simulink model "TV_FLC_V3"  (R2026b)
settings: Solver=VariableStepAuto
model mask{MotorT=Control.MotorTrq, Gr=Control.GearRatio, MotorW=Control.MotorW, rwheel=Control.WheelRad, tr=Control.RearTrack, a=Control.FrontTrackToCG, a_cop=Control.FrontTrackToCoP, Af=Control.FrontalArea, cd=Control.LiftCoef, Value=Control.GravitationalAcc, ro=Control.AirDensity, m=Control.Mass, h_CG=Control.CGHeight, L=Control.Wheelbase, StrWhlR=Control.StrWheelRatio, Ku=Control.UndersteerGradient, F=Control.F, Slip_Ctrl_Kp=Control.Proportional_P, Slip_Ctrl_Ki=Control.Integral_I, Slip_Ctrl_Kd=Control.Derivative_D, Slip_Ctrl_Kn=Control.Filter_N, Load_Ref=Control.LoadRef, Slip_Ref=Control.SlipRef, FIS=Control.FuzzySystem, vx_th=Control.ActivationVelocity, Tmax=max(Control.MotorTrq), C_alpha_F=Control.CalphaF, Slip_Steer_th=10, Kp_TV_Yaw=Control.Kp_Yaw, Kp_TV_Beta=Control.Kp_beta}
  mask prompts: MotorT "Motor Torque:"; Gr "Gear Ratio:"; MotorW "Motor RPM:"; rwheel "Wheel Radius:"; tr "Rear Track:"; a "Front Track to CG:"; a_cop "Front Track to CoP"; Af "Frontal Area:"; cd "Lift Coef:"; Value "Simulink:blkprm_prompts:ConstConstValue"; ro "Air Density:"; m "Mass:"; h_CG "CG Height:"; L "Wheelbase:"; StrWhlR "Steering Wheel Ratio:"; Ku "Understeer Gradient:"; F "Moment to Torque"; Slip_Ctrl_Kp "Simulink:masks:ProportionalP_MP"; Slip_Ctrl_Ki "Simulink:masks:IntegralI_MP"; Slip_Ctrl_Kd "Simulink:masks:DerivativeD_MP"; Slip_Ctrl_Kn "Filter (N):"; Load_Ref "Reference Load Table:"; Slip_Ref "Reference Slip Table:"; FIS "Fuzzy Inference System"; vx_th "Activation Velocity:"; Tmax "Max Torque"; C_alpha_F "Front Cornering Stiffness:"; Slip_Steer_th "Steering activation threshold:"; Kp_TV_Yaw "TV Yaw factor:"; Kp_TV_Beta "TV Beta factor:"
values from neighbouring files (symbols this model uses):
  a = -Vehicle.Chassis.Body.sCG.Value(1)    [sm_car_controlparam_FLCDYC_V3.m]
  Gr = 1/Vehicle.Powertrain.Driveline.Gearbox.ratio.Value    [sm_car_controlparam_FLCDYC_V3.m]
  L = 1.578    [sm_car_controlparam_FLCDYC_V3.m]
  rwheel = 0.263    [sm_car_controlparam_FLCDYC_V3.m]
  tr = Vehicle.Chassis.Body.TrackRear.Value    [sm_car_controlparam_FLCDYC_V3.m]
undefined symbols (not defined in the file or in its folder): dspblkCoreblockFVToolHelper, gcbh
libraries: simulink x5, sl_discontinuities x3, slpidlib x2, fuzblock x1
settings Model: Creator=andrei  LastModifiedBy=andrei

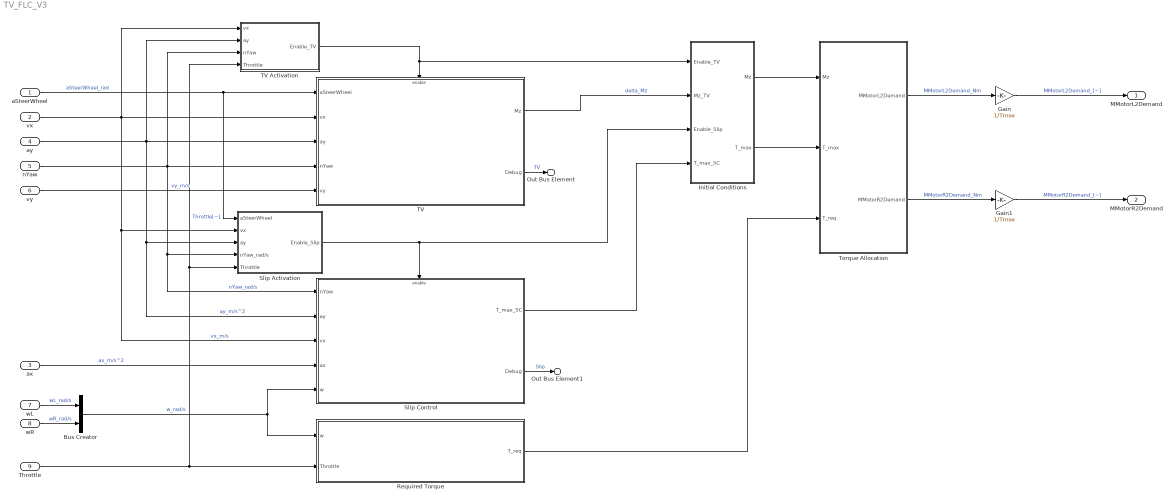
== system TV_FLC_V3 ==
  aSteerWheel : Inport  OutDataTypeStr=single  PortDimensions=1  SampleTime=0.003
  vx : Inport  Port=2  OutDataTypeStr=single  PortDimensions=1  SampleTime=0.003
  ax : Inport  Port=3  OutDataTypeStr=single  PortDimensions=1  SampleTime=0.003
  ay : Inport  Port=4  OutDataTypeStr=single  PortDimensions=1  SampleTime=0.003
  nYaw : Inport  Port=5  OutDataTypeStr=single  PortDimensions=1  SampleTime=0.003
  vy : Inport  Port=6  OutDataTypeStr=single  PortDimensions=1  SampleTime=0.003
  wL : Inport  Port=7  OutDataTypeStr=single  PortDimensions=1  SampleTime=0.003
  wR : Inport  Port=8  OutDataTypeStr=single  PortDimensions=1  SampleTime=0.003
  Throttle : Inport  Port=9  OutDataTypeStr=single  PortDimensions=1  SampleTime=0.003
  Bus Creator : BusCreator  Inputs=2
  Gain : Gain  Gain=1/Tmax
  Gain1 : Gain  Gain=1/Tmax
  Initial Conditions : Subsystem
  Required Torque : Subsystem
  Slip Activation : Subsystem
  Slip Control : Subsystem
  TV : Subsystem
  TV Activation : Subsystem
  Torque Allocation : Subsystem
  MMotorL2Demand : Outport  OutDataTypeStr=single  PortDimensions=1  SampleTime=0.003
  MMotorR2Demand : Outport  Port=2  OutDataTypeStr=single  PortDimensions=1  SampleTime=0.003
  Out Bus Element : Outport  Port=3  PortName=Debug  Element=TV
  Out Bus Element1 : Outport  Port=3  PortName=Debug  Element=Slip
  wires:
  Gain1/1 -> MMotorR2Demand/1  "MMotorR2Demand_[~]"
  Torque Allocation/2(MMotorR2Demand) -> Gain1/1  "MMotorR2Demand_Nm"
  vy/1 -> TV/5(vy)  "vy_m/s"
  Gain/1 -> MMotorL2Demand/1  "MMotorL2Demand_[~]"
  Slip Control/1(T_max_SC) -> Initial Conditions/4(T_max_SC)
  Slip Control/2(Debug) -> Out Bus Element1/1  "Slip"
  ax/1 -> Slip Control/4(ax)  "ax_m/s^2"
  Initial Conditions/2(T_max) -> Torque Allocation/2(T_max)
  wL/1 -> Bus Creator/1  "wL_rad/s"
  TV/1(Mz) -> Initial Conditions/2(Mz_TV)  "delta_Mz"
  Torque Allocation/1(MMotorL2Demand) -> Gain/1  "MMotorL2Demand_Nm"
  TV Activation/1(Enable_TV) -> Initial Conditions/1(Enable_TV), TV/Enable
  TV/2(Debug) -> Out Bus Element/1  "TV"
  wR/1 -> Bus Creator/2  "wR_rad/s"
  Bus Creator/1 -> Required Torque/1(w), Slip Control/5(w)  "w_rad/s"
  Initial Conditions/1(Mz) -> Torque Allocation/1(Mz)
  Required Torque/1(T_req) -> Torque Allocation/3(T_req)
  vx/1 -> TV Activation/1(vx), Slip Activation/2(vx), Slip Control/3(vx), TV/2(vx)  "vx_m/s"
  nYaw/1 -> TV Activation/3(nYaw), TV/4(nYaw), Slip Activation/4(nYaw_rad/s), Slip Control/1(nYaw)  "nYaw_rad/s"
  Throttle/1 -> TV Activation/4(Throttle), Slip Activation/5(Throttle), Required Torque/2(Throttle)  "Throttle[~]"
  aSteerWheel/1 -> Slip Activation/1(aSteerWheel), TV/1(aSteerWheel)  "aSteerWheel_rad"
  ay/1 -> Slip Activation/3(ay), Slip Control/2(ay), TV Activation/2(ay), TV/3(ay)  "ay_m/s^2"
  Slip Activation/1(Enable_Slip) -> Slip Control/Enable, Initial Conditions/3(Enable_Slip)

== system TV_FLC_V3/Initial Conditions ==
  Enable_TV : Inport
  Mz_TV : Inport  Port=2
  Enable_Slip : Inport  Port=3
  T_max_SC : Inport  Port=4
  Bus Creator1 : BusCreator  Inputs=2
  Constant : Constant  Value=Tmax  OutDataTypeStr=single
  Constant1 : Constant  Value=Tmax  OutDataTypeStr=single
  Constant2 : Constant  Value=0  OutDataTypeStr=single
  Switch : Switch  Criteria=u2 ~= 0  SaturateOnIntegerOverflow=off  InputSameDT=off
  Switch1 : Switch  Criteria=u2 ~= 0  SaturateOnIntegerOverflow=off  InputSameDT=off
  Mz : Outport
  T_max : Outport  Port=2
  wires:
  Enable_Slip/1 -> Switch/2
  Enable_TV/1 -> Switch1/2
  Constant1/1 -> Bus Creator1/2  "Tmax_rr_Nm"
  Switch/1 -> T_max/1
  Bus Creator1/1 -> Switch/3
  T_max_SC/1 -> Switch/1
  Constant/1 -> Bus Creator1/1  "Tmax_rl_Nm"
  Mz_TV/1 -> Switch1/1
  Constant2/1 -> Switch1/3  "Mz"
  Switch1/1 -> Mz/1

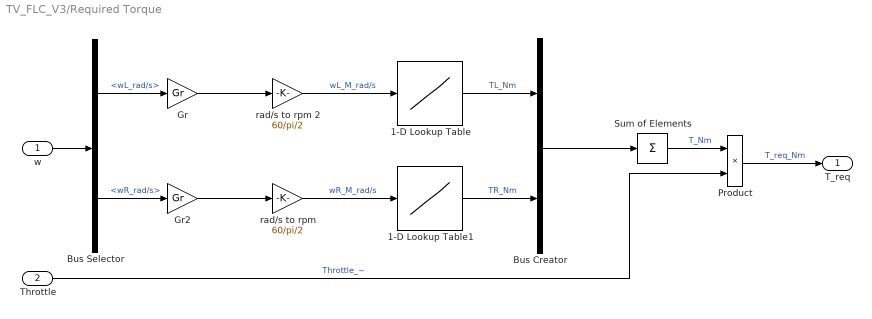
== system TV_FLC_V3/Required Torque ==
  w : Inport
  Throttle : Inport  Port=2
  1-D Lookup Table : Lookup_n-D  NumberOfTableDimensions=1  BreakpointsForDimension1=MotorW  Table=MotorT  InternalRulePriority=Speed  RndMeth=Simplest
  1-D Lookup Table1 : Lookup_n-D  NumberOfTableDimensions=1  BreakpointsForDimension1=MotorW  Table=MotorT  InternalRulePriority=Speed  RndMeth=Simplest
  Bus Creator : BusCreator  Inputs=2
  Bus Selector : BusSelector  OutputSignals=wL_rad/s,wR_rad/s
  Gr : Gain  Gain=Gr
  Gr2 : Gain  Gain=Gr
  Product : Product
  Sum of Elements : Sum  Inputs=+
  rad/s to rpm : Gain  Gain=60/pi/2
  rad/s to rpm 2 : Gain  Gain=60/pi/2
  T_req : Outport
  wires:
  w/1 -> Bus Selector/1
  Sum of Elements/1 -> Product/1  "T_Nm"
  1-D Lookup Table1/1 -> Bus Creator/2  "TR_Nm"
  Throttle/1 -> Product/2  "Throttle_~"
  rad/s to rpm/1 -> 1-D Lookup Table1/1  "wR_M_rad/s"
  Bus Selector/1 -> Gr/1  "<wL_rad/s>"
  Product/1 -> T_req/1  "T_req_Nm"
  Bus Selector/2 -> Gr2/1  "<wR_rad/s>"
  rad/s to rpm 2/1 -> 1-D Lookup Table/1  "wL_M_rad/s"
  1-D Lookup Table/1 -> Bus Creator/1  "TL_Nm"
  Bus Creator/1 -> Sum of Elements/1
  Gr/1 -> rad/s to rpm 2/1
  Gr2/1 -> rad/s to rpm/1

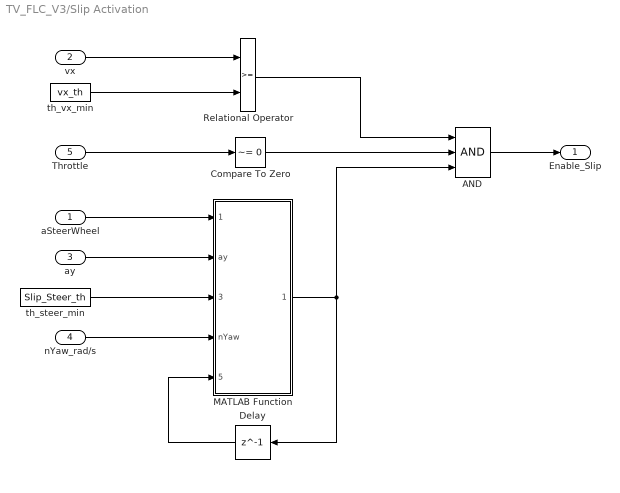
== system TV_FLC_V3/Slip Activation ==
  aSteerWheel : Inport
  vx : Inport  Port=2
  ay : Inport  Port=3
  nYaw_rad/s : Inport  Port=4
  Throttle : Inport  Port=5
  AND : Logic  Inputs=3  AllPortsSameDT=off  OutDataTypeStr=boolean
  Compare To Zero : simulink/Logic and Bit Operations/Compare To Zero  relop=~=  OutDataTypeStr=boolean
  Delay : Delay  DelayLength=1
  MATLAB Function : MATLAB Function  TreatAsAtomicUnit=on
  Relational Operator : RelationalOperator  OutDataTypeStr=boolean  RndMeth=Simplest  InputSameDT=off
  th_steer_min : Constant  Value=Slip_Steer_th
  th_vx_min : Constant  Value=vx_th
  Enable_Slip : Outport
  wires:
  Compare To Zero/1 -> AND/2
  AND/1 -> Enable_Slip/1
  Throttle/1 -> Compare To Zero/1
  th_vx_min/1 -> Relational Operator/2
  vx/1 -> Relational Operator/1
  Relational Operator/1 -> AND/1
  aSteerWheel/1 -> MATLAB Function/1(aSteerWheel)
  th_steer_min/1 -> MATLAB Function/3(steer_th)
  ay/1 -> MATLAB Function/2(ay)
  nYaw_rad/s/1 -> MATLAB Function/4(nYaw)
  MATLAB Function/1(slip_active) -> Delay/1, AND/3
  Delay/1 -> MATLAB Function/5(slip_active_previous)

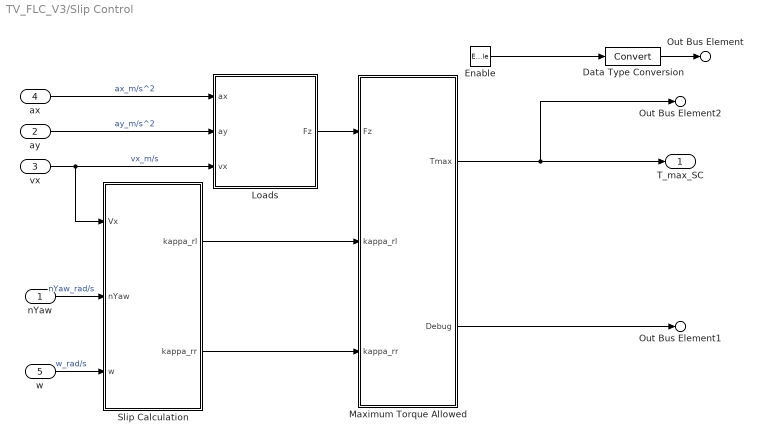
== system TV_FLC_V3/Slip Control ==
  nYaw : Inport
  ay : Inport  Port=2
  vx : Inport  Port=3
  ax : Inport  Port=4
  w : Inport  Port=5
  Enable : EnablePort  StatesWhenEnabling=reset  ShowOutputPort=on  OutDataTypeStr=boolean
  Data Type Conversion : DataTypeConversion  SaturateOnIntegerOverflow=off  RndMeth=Floor
  Loads : Subsystem
  Maximum Torque Allowed : Subsystem
  Slip Calculation : Subsystem
  T_max_SC : Outport  OutputWhenDisabled=reset  InitialOutput=Tmax
  Out Bus Element : Outport  Port=2  PortName=Debug  Element=State
  Out Bus Element1 : Outport  Port=2  PortName=Debug  Element=Controller
  Out Bus Element2 : Outport  Port=2  PortName=Debug  Element=TmaxOut
  wires:
  Maximum Torque Allowed/2(Debug) -> Out Bus Element1/1
  Enable/1 -> Data Type Conversion/1
  w/1 -> Slip Calculation/3(w)  "w_rad/s"
  nYaw/1 -> Slip Calculation/2(nYaw)  "nYaw_rad/s"
  ax/1 -> Loads/1(ax)  "ax_m/s^2"
  Loads/1(Fz) -> Maximum Torque Allowed/1(Fz)
  ay/1 -> Loads/2(ay)  "ay_m/s^2"
  Slip Calculation/2(kappa_rr) -> Maximum Torque Allowed/3(kappa_rr)
  vx/1 -> Loads/3(vx), Slip Calculation/1(Vx)  "vx_m/s"
  Slip Calculation/1(kappa_rl) -> Maximum Torque Allowed/2(kappa_rl)
  Data Type Conversion/1 -> Out Bus Element/1
  Maximum Torque Allowed/1(Tmax) -> Out Bus Element2/1, T_max_SC/1

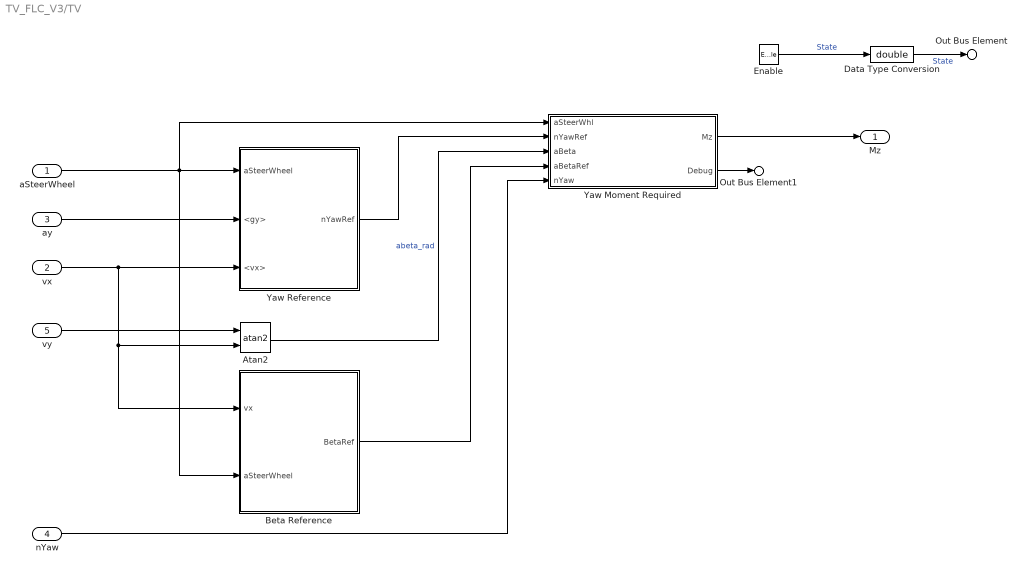
== system TV_FLC_V3/TV ==
  aSteerWheel : Inport
  vx : Inport  Port=2
  ay : Inport  Port=3
  nYaw : Inport  Port=4
  vy : Inport  Port=5
  Enable : EnablePort  StatesWhenEnabling=reset  ShowOutputPort=on  OutDataTypeStr=boolean
  Atan2 : Trigonometry  Operator=atan2
  Beta Reference : Subsystem
  Data Type Conversion : DataTypeConversion  OutDataTypeStr=double  SaturateOnIntegerOverflow=off  RndMeth=Floor
  Yaw Moment Required : Subsystem
  Yaw Reference : Subsystem
  Mz : Outport  OutputWhenDisabled=reset  InitialOutput=0
  Out Bus Element : Outport  Port=2  PortName=Debug  Element=State
  Out Bus Element1 : Outport  Port=2  PortName=Debug  Element=Controller
  wires:
  Yaw Moment Required/2(Debug) -> Out Bus Element1/1
  Data Type Conversion/1 -> Out Bus Element/1  "State"
  vy/1 -> Atan2/1
  Beta Reference/1(BetaRef) -> Yaw Moment Required/4(aBetaRef)
  Yaw Reference/1(nYawRef) -> Yaw Moment Required/2(nYawRef)
  ay/1 -> Yaw Reference/2(<gy>)
  nYaw/1 -> Yaw Moment Required/5(nYaw)
  vx/1 -> Yaw Reference/3(<vx>), Atan2/2, Beta Reference/1(vx)
  aSteerWheel/1 -> Yaw Reference/1(aSteerWheel), Yaw Moment Required/1(aSteerWhl), Beta Reference/2(aSteerWheel)
  Atan2/1 -> Yaw Moment Required/3(aBeta)  "abeta_rad"
  Yaw Moment Required/1(Mz) -> Mz/1
  Enable/1 -> Data Type Conversion/1  "State"

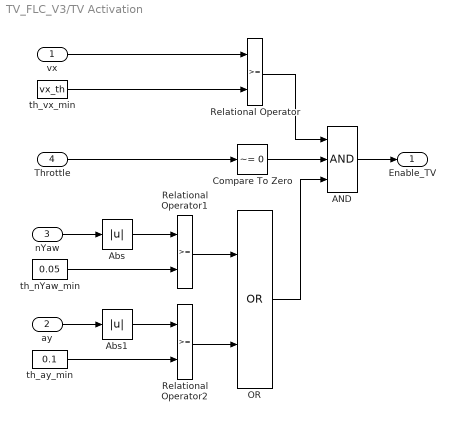
== system TV_FLC_V3/TV Activation ==
  vx : Inport
  ay : Inport  Port=2
  nYaw : Inport  Port=3
  Throttle : Inport  Port=4
  AND : Logic  Inputs=3  AllPortsSameDT=off  OutDataTypeStr=boolean
  Abs : Abs  SaturateOnIntegerOverflow=off
  Abs1 : Abs  SaturateOnIntegerOverflow=off
  Compare To Zero : simulink/Logic and Bit Operations/Compare To Zero  relop=~=  OutDataTypeStr=boolean
  OR : Logic  Operator=OR  AllPortsSameDT=off  OutDataTypeStr=boolean
  Relational Operator : RelationalOperator  OutDataTypeStr=boolean  RndMeth=Simplest  InputSameDT=off
  Relational Operator1 : RelationalOperator  OutDataTypeStr=boolean  RndMeth=Simplest  InputSameDT=off
  Relational Operator2 : RelationalOperator  OutDataTypeStr=boolean  RndMeth=Simplest  InputSameDT=off
  th_ay_min : Constant  Value=0.1  OutDataTypeStr=single
  th_nYaw_min : Constant  Value=0.05  OutDataTypeStr=single
  th_vx_min : Constant  Value=vx_th
  Enable_TV : Outport
  wires:
  ay/1 -> Abs1/1
  th_nYaw_min/1 -> Relational Operator1/2
  Abs1/1 -> Relational Operator2/1
  Throttle/1 -> Compare To Zero/1
  Abs/1 -> Relational Operator1/1
  vx/1 -> Relational Operator/1
  nYaw/1 -> Abs/1
  th_ay_min/1 -> Relational Operator2/2
  th_vx_min/1 -> Relational Operator/2
  Relational Operator1/1 -> OR/1
  Relational Operator2/1 -> OR/2
  Relational Operator/1 -> AND/1
  Compare To Zero/1 -> AND/2
  OR/1 -> AND/3
  AND/1 -> Enable_TV/1

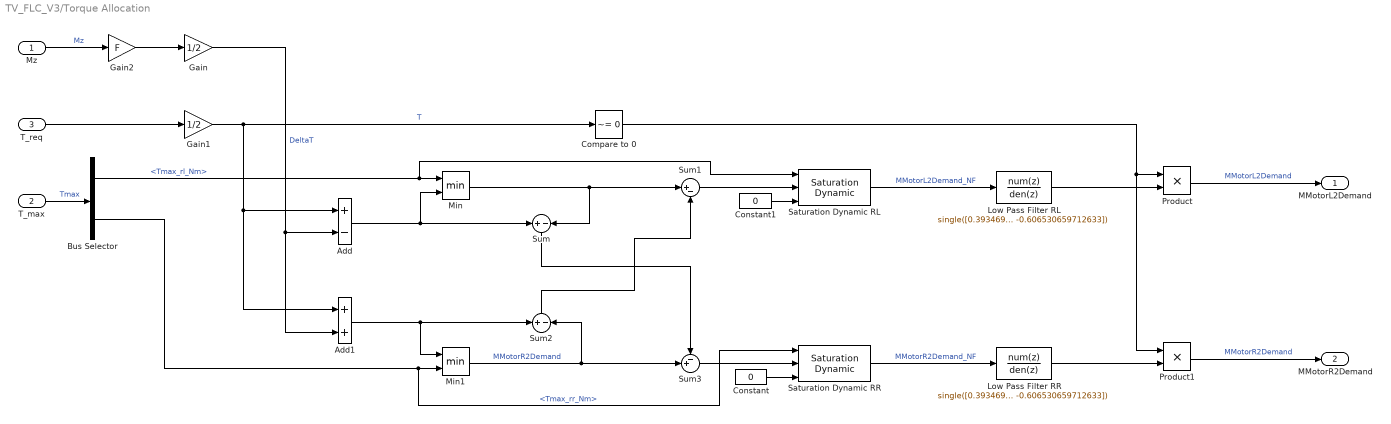
== system TV_FLC_V3/Torque Allocation ==
  Mz : Inport
  T_max : Inport  Port=2
  T_req : Inport  Port=3
  Add : Sum  Inputs=+-
  Add1 : Sum
  Bus Selector : BusSelector  OutputSignals=Tmax_rl_Nm,Tmax_rr_Nm
  "Compare to 0 " : simulink/Logic and Bit Operations/Compare To Constant  relop=~=  const=0  OutDataTypeStr=boolean
  Constant : Constant  Value=0
  Constant1 : Constant  Value=0
  Gain : Gain  Gain=1/2
  Gain1 : Gain  Gain=1/2
  Gain2 : Gain  Gain=F
  Low Pass Filter RL : DiscreteTransferFcn  LoadFcn=dspblkCoreblockFVToolHelper(gcbh,'load');  Numerator=single([0.393469340287367])  Denominator=single([1 -0.606530659712633])
      settings: CopyFcn=dspblkCoreblockFVToolHelper(gcbh,'copy');  DeleteFcn=dspblkCoreblockFVToolHelper(gcbh,'close');  ModelCloseFcn=dspblkCoreblockFVToolHelper(gcbh,'close');  PreSaveFcn=dspblkCoreblockFVToolHelper(gcbh,'presave');  PostSaveFcn=dspblkCoreblockFVToolHelper(gcbh,'postsave');  CloseFcn=dspblkCoreblockFVToolHelper(gcbh,'close');
  Low Pass Filter RR : DiscreteTransferFcn  LoadFcn=dspblkCoreblockFVToolHelper(gcbh,'load');  Numerator=single([0.393469340287367])  Denominator=single([1 -0.606530659712633])
      settings: CopyFcn=dspblkCoreblockFVToolHelper(gcbh,'copy');  DeleteFcn=dspblkCoreblockFVToolHelper(gcbh,'close');  ModelCloseFcn=dspblkCoreblockFVToolHelper(gcbh,'close');  PreSaveFcn=dspblkCoreblockFVToolHelper(gcbh,'presave');  PostSaveFcn=dspblkCoreblockFVToolHelper(gcbh,'postsave');  CloseFcn=dspblkCoreblockFVToolHelper(gcbh,'close');
  Min : MinMax  Inputs=2
  Min1 : MinMax  Inputs=2
  Product : Product
  Product1 : Product
  Saturation Dynamic RL : sl_discontinuities/Saturation Dynamic  OutMin=[]  OutMax=[]  OutDataTypeStr=single  OutDataType=fixdt(1, 16)  OutScaling=2^-10  DoSatur=off
      settings: LibrarySourceBlock=|
      | simulink/Discontinuities/Saturation
      | Dynamic
  Saturation Dynamic RR : sl_discontinuities/Saturation Dynamic  OutMin=[]  OutMax=[]  OutDataTypeStr=single  OutDataType=fixdt(1, 16)  OutScaling=2^-10  DoSatur=off
      settings: LibrarySourceBlock=|
      | simulink/Discontinuities/Saturation
      | Dynamic
  Sum : Sum  Inputs=+|-
  Sum1 : Sum  Inputs=|+-
  Sum2 : Sum  Inputs=+|-
  Sum3 : Sum  Inputs=-+|
  MMotorL2Demand : Outport
  MMotorR2Demand : Outport  Port=2
  wires:
  Constant1/1 -> Saturation Dynamic RL/3
  Constant/1 -> Saturation Dynamic RR/3
  Product1/1 -> MMotorR2Demand/1  "MMotorR2Demand"
  Low Pass Filter RR/1 -> Product1/2
  Saturation Dynamic RR/1 -> Low Pass Filter RR/1  "MMotorR2Demand_NF"
  Product/1 -> MMotorL2Demand/1  "MMotorL2Demand"
  Low Pass Filter RL/1 -> Product/2
  "Compare to 0 "/1 -> Product1/1, Product/1
  Gain1/1 -> Add/1, Add1/1, "Compare to 0 "/1  "T"
  Sum/1 -> Sum3/1
  Sum2/1 -> Sum1/2
  Add1/1 -> Min1/1, Sum2/1
  Add/1 -> Min/2, Sum/1
  Bus Selector/2 -> Saturation Dynamic RR/1, Min1/2  "<Tmax_rr_Nm>"
  Bus Selector/1 -> Min/1, Saturation Dynamic RL/1  "<Tmax_rl_Nm>"
  T_max/1 -> Bus Selector/1  "Tmax"
  Min1/1 -> Sum3/2, Sum2/2  "MMotorR2Demand"
  Min/1 -> Sum/2, Sum1/1
  Mz/1 -> Gain2/1  "Mz"
  T_req/1 -> Gain1/1
  Gain/1 -> Add/2, Add1/2  "DeltaT"
  Gain2/1 -> Gain/1
  Sum1/1 -> Saturation Dynamic RL/2
  Sum3/1 -> Saturation Dynamic RR/2
  Saturation Dynamic RL/1 -> Low Pass Filter RL/1  "MMotorL2Demand_NF"

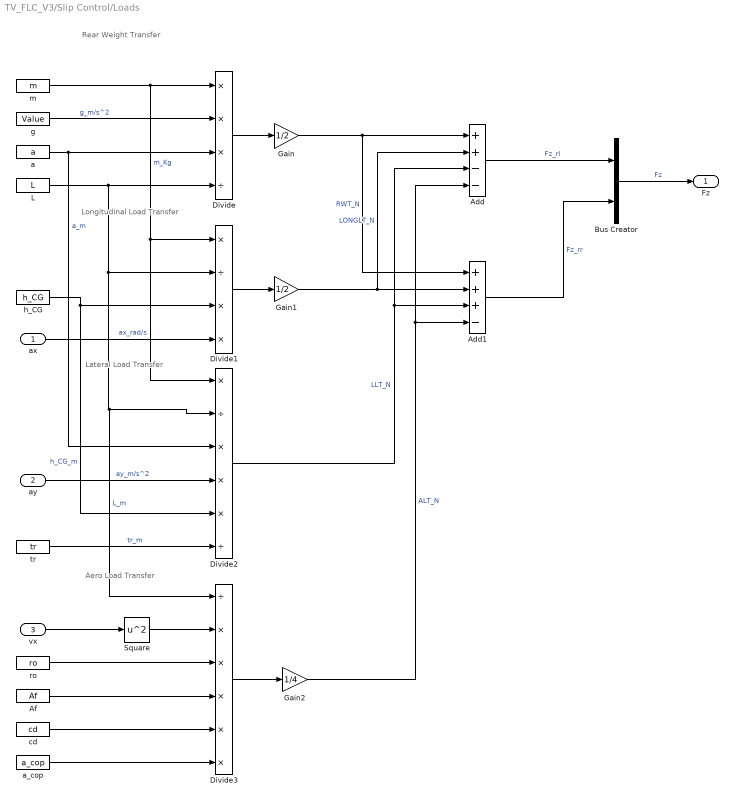
== system TV_FLC_V3/Slip Control/Loads ==
  note: Rear Weight Transfer
  note: Longitudinal Load Transfer
  note: Lateral Load Transfer
  note: Aero Load Transfer
  ax : Inport
  ay : Inport  Port=2
  vx : Inport  Port=3
  Add : Sum  Inputs=++--
  Add1 : Sum  Inputs=+++-
  Af : Constant  Value=Af  OutDataTypeStr=single
  Bus Creator : BusCreator  Inputs=2
  Divide : Product  Inputs=***/
  Divide1 : Product  Inputs=*/**
  Divide2 : Product  Inputs=*/***/
  Divide3 : Product  Inputs=/*****
  Gain : Gain  Gain=1/2
  Gain1 : Gain  Gain=1/2
  Gain2 : Gain  Gain=1/4
  L : Constant  Value=L  OutDataTypeStr=single
  Square : Math  Operator=square
  a : Constant  Value=a  OutDataTypeStr=single
  a_cop : Constant  Value=a_cop  OutDataTypeStr=single
  cd : Constant  Value=cd  OutDataTypeStr=single
  g : Constant  Value=Value  OutDataTypeStr=single
  h_CG : Constant  Value=h_CG  OutDataTypeStr=single
  m : Constant  Value=m  OutDataTypeStr=single
  ro : Constant  Value=ro  OutDataTypeStr=single
  tr : Constant  Value=tr  OutDataTypeStr=single
  Fz : Outport
  wires:
  a_cop/1 -> Divide3/6
  cd/1 -> Divide3/5
  Af/1 -> Divide3/4
  ro/1 -> Divide3/3
  Divide3/1 -> Gain2/1
  Bus Creator/1 -> Fz/1  "Fz"
  Add1/1 -> Bus Creator/2  "Fz_rr"
  Add/1 -> Bus Creator/1  "Fz_rl"
  Divide2/1 -> Add1/3, Add/3  "LLT_N"
  tr/1 -> Divide2/6  "tr_m"
  ay/1 -> Divide2/4  "ay_m/s^2"
  Gain1/1 -> Add1/2, Add/2  "LONGLT_N"
  Divide1/1 -> Gain1/1
  ax/1 -> Divide1/4  "ax_rad/s"
  h_CG/1 -> Divide1/3, Divide2/5  "h_CG_m"
  Gain2/1 -> Add1/4, Add/4  "ALT_N"
  Gain/1 -> Add1/1, Add/1  "RWT_N"
  Square/1 -> Divide3/2
  vx/1 -> Square/1
  Divide/1 -> Gain/1
  L/1 -> Divide/4, Divide1/2, Divide2/2, Divide3/1  "L_m"
  a/1 -> Divide2/3, Divide/3  "a_m"
  g/1 -> Divide/2  "g_m/s^2"
  m/1 -> Divide2/1, Divide1/1, Divide/1  "m_Kg"

== system TV_FLC_V3/Slip Control/Maximum Torque Allowed ==
  Fz : Inport
  kappa_rl : Inport  Port=2
  kappa_rr : Inport  Port=3
  Bus Creator : BusCreator  Inputs=2
  Bus Selector : BusSelector  OutputSignals=Fz_rl,Fz_rr
  Slip Correction Left : Subsystem
  Slip Correction Right : Subsystem
  Tmax : Outport  OutDataTypeStr=single
  Out Bus Element : Outport  Port=2  PortName=Debug  Element=PID_rl
  Out Bus Element1 : Outport  Port=2  PortName=Debug  Element=PID_rr
  wires:
  Slip Correction Right/1(Debug) -> Out Bus Element1/1
  Slip Correction Left/2(Debug) -> Out Bus Element/1
  Slip Correction Right/2(Tmax_rr) -> Bus Creator/2  "Tmax_rr_Nm"
  Slip Correction Left/1(Tmax_rl) -> Bus Creator/1  "Tmax_rl_Nm"
  kappa_rl/1 -> Slip Correction Left/1(kappa_rl)
  kappa_rr/1 -> Slip Correction Right/2(kappa_rr)
  Fz/1 -> Bus Selector/1
  Bus Selector/1 -> Slip Correction Left/2(Fz_rl)  "<Fz_rl>"
  Bus Selector/2 -> Slip Correction Right/1(Fz_rl)  "<Fz_rr>"
  Bus Creator/1 -> Tmax/1

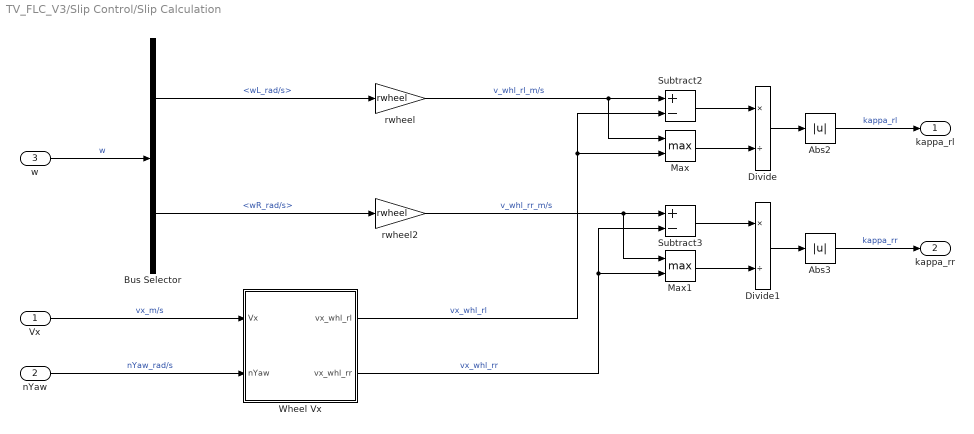
== system TV_FLC_V3/Slip Control/Slip Calculation ==
  Vx : Inport
  nYaw : Inport  Port=2
  w : Inport  Port=3
  Abs2 : Abs  SaturateOnIntegerOverflow=off
  Abs3 : Abs  SaturateOnIntegerOverflow=off
  Bus Selector : BusSelector  OutputSignals=wL_rad/s,wR_rad/s
  Divide : Product  Inputs=*/
  Divide1 : Product  Inputs=*/
  Max : MinMax  Function=max  Inputs=2
  Max1 : MinMax  Function=max  Inputs=2
  Subtract2 : Sum  Inputs=+-
  Subtract3 : Sum  Inputs=+-
  Wheel Vx : Subsystem
  rwheel : Gain  Gain=rwheel
  rwheel2 : Gain  Gain=rwheel
  kappa_rl : Outport
  kappa_rr : Outport  Port=2
  wires:
  Max1/1 -> Divide1/2
  Divide1/1 -> Abs3/1
  Max/1 -> Divide/2
  Divide/1 -> Abs2/1
  Subtract3/1 -> Divide1/1
  Wheel Vx/2(vx_whl_rr) -> Max1/2, Subtract3/2  "vx_whl_rr"
  Subtract2/1 -> Divide/1
  Abs2/1 -> kappa_rl/1  "kappa_rl"
  Wheel Vx/1(vx_whl_rl) -> Max/2, Subtract2/2  "vx_whl_rl"
  Abs3/1 -> kappa_rr/1  "kappa_rr"
  nYaw/1 -> Wheel Vx/2(nYaw)  "nYaw_rad/s"
  rwheel2/1 -> Subtract3/1, Max1/1  "v_whl_rr_m/s"
  rwheel/1 -> Subtract2/1, Max/1  "v_whl_rl_m/s"
  w/1 -> Bus Selector/1  "w"
  Vx/1 -> Wheel Vx/1(Vx)  "vx_m/s"
  Bus Selector/2 -> rwheel2/1  "<wR_rad/s>"
  Bus Selector/1 -> rwheel/1  "<wL_rad/s>"

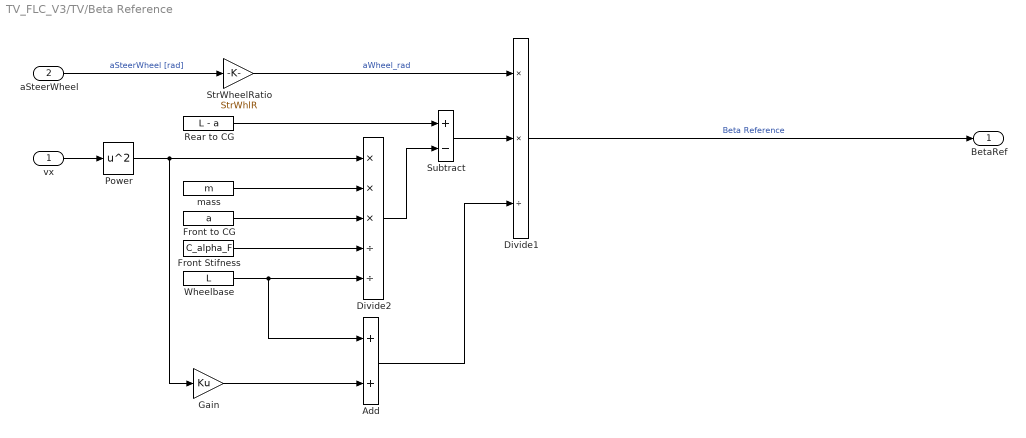
== system TV_FLC_V3/TV/Beta Reference ==
  vx : Inport
  aSteerWheel : Inport  Port=2
  Add : Sum
  Divide1 : Product  Inputs=**/
  Divide2 : Product  Inputs=***//
  Front Stifness : Constant  Value=C_alpha_F  OutDataTypeStr=single
  Front to CG : Constant  Value=a  OutDataTypeStr=single
  Gain : Gain  Gain=Ku  ParamDataTypeStr=single
  Power : Math  Operator=square
  Rear to CG : Constant  Value=L - a  OutDataTypeStr=single
  StrWheelRatio : Gain  Gain=StrWhlR
  Subtract : Sum  Inputs=+-
  Wheelbase : Constant  Value=L  OutDataTypeStr=single
  mass : Constant  Value=m  OutDataTypeStr=single
  BetaRef : Outport
  wires:
  Subtract/1 -> Divide1/2
  Divide2/1 -> Subtract/2
  Rear to CG/1 -> Subtract/1
  Front to CG/1 -> Divide2/3
  mass/1 -> Divide2/2
  Front Stifness/1 -> Divide2/4
  Wheelbase/1 -> Divide2/5, Add/1
  aSteerWheel/1 -> StrWheelRatio/1  "aSteerWheel [rad]"
  vx/1 -> Power/1
  Divide1/1 -> BetaRef/1  "Beta Reference"
  Power/1 -> Divide2/1, Gain/1
  Gain/1 -> Add/2
  Add/1 -> Divide1/3
  StrWheelRatio/1 -> Divide1/1  "aWheel_rad"

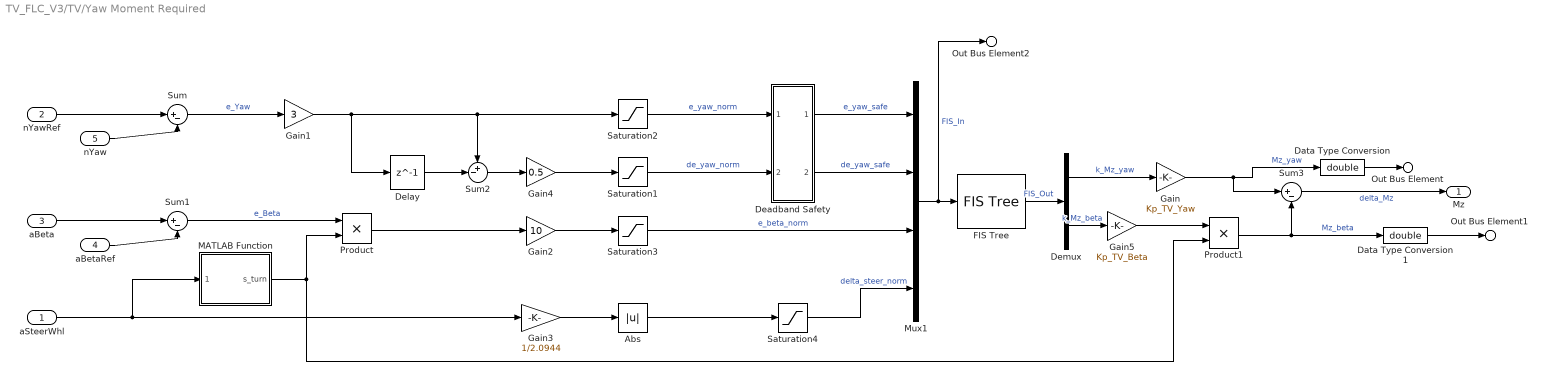
== system TV_FLC_V3/TV/Yaw Moment Required ==
  aSteerWhl : Inport  OutDataTypeStr=single
  nYawRef : Inport  Port=2  OutDataTypeStr=single
  aBeta : Inport  Port=3  OutDataTypeStr=single
  aBetaRef : Inport  Port=4  OutDataTypeStr=single
  nYaw : Inport  Port=5  OutDataTypeStr=single
  Abs : Abs  SaturateOnIntegerOverflow=off
  Data Type Conversion : DataTypeConversion  OutDataTypeStr=double  SaturateOnIntegerOverflow=off  RndMeth=Floor
  Data Type Conversion1 : DataTypeConversion  OutDataTypeStr=double  SaturateOnIntegerOverflow=off  RndMeth=Floor
  Deadband Safety : Subsystem
  Delay : Delay  DelayLength=1  InputProcessing=Columns as channels (frame based)
  Demux : Demux  Outputs=2
  FIS Tree : fuzblock/FIS Tree  FIS=FIS  OutputSampleNumber=101  DataType=single  UseLookupTable=off  NumBreakpoints=10  SimulateUsing=Code generation  OutOfRangeInputValueMessage=warning  NoRuleFiredMessage=warning  EmptyOutputFuzzySetMessage=warning
  Gain : Gain  Gain=Kp_TV_Yaw  OutDataTypeStr=single
  Gain1 : Gain  Gain=3
  Gain2 : Gain  Gain=10  OutDataTypeStr=single
  Gain3 : Gain  Gain=1/2.0944  OutDataTypeStr=single
  Gain4 : Gain  Gain=0.5
  Gain5 : Gain  Gain=Kp_TV_Beta  OutDataTypeStr=single
  MATLAB Function : MATLAB Function  TreatAsAtomicUnit=on  mask{delta_th=Slip_Steer_th/2}
      mask prompts: delta_th "Steering Th"
  Mux1 : Mux
  Product : Product
  Product1 : Product
  Saturation1 : Saturate  UpperLimit=1  LowerLimit=-1
  Saturation2 : Saturate  UpperLimit=1  LowerLimit=-1
  Saturation3 : Saturate  UpperLimit=1  LowerLimit=-1  ZeroCross=off
  Saturation4 : Saturate  UpperLimit=1  LowerLimit=0  ZeroCross=off
  Sum : Sum  Inputs=|+-
  Sum1 : Sum  Inputs=|+-
  Sum2 : Sum  Inputs=+-|
  Sum3 : Sum  Inputs=|+-  OutDataTypeStr=Inherit: Same as first input
  Mz : Outport  OutDataTypeStr=single
  Out Bus Element : Outport  Port=2  PortName=Debug  Element=Mz_yaw
  Out Bus Element1 : Outport  Port=2  PortName=Debug  Element=Mz_Beta
  Out Bus Element2 : Outport  Port=2  PortName=Debug  Element=FIS_In
  wires:
  Deadband Safety/2(de_yaw_safe) -> Mux1/2  "de_yaw_safe"
  Deadband Safety/1(e_yaw_safe) -> Mux1/1  "e_yaw_safe"
  Saturation1/1 -> Deadband Safety/2(de_yaw_norm)  "de_yaw_norm"
  Saturation2/1 -> Deadband Safety/1(e_yaw_norm)  "e_yaw_norm"
  Abs/1 -> Saturation4/1
  Product1/1 -> Data Type Conversion1/1, Sum3/2  "Mz_beta"
  Gain5/1 -> Product1/1
  Sum3/1 -> Mz/1  "delta_Mz"
  Demux/2 -> Gain5/1  "k_Mz_beta"
  Demux/1 -> Gain/1  "k_Mz_yaw"
  Product/1 -> Gain2/1
  MATLAB Function/1(s_turn) -> Product/2, Product1/2
  Gain4/1 -> Saturation1/1
  Saturation4/1 -> Mux1/4  "delta_steer_norm"
  Saturation3/1 -> Mux1/3  "e_beta_norm"
  Gain3/1 -> Abs/1
  Gain2/1 -> Saturation3/1
  Gain1/1 -> Saturation2/1, Sum2/1, Delay/1
  aSteerWhl/1 -> MATLAB Function/1(delta_SW), Gain3/1
  aBetaRef/1 -> Sum1/2
  aBeta/1 -> Sum1/1
  Sum1/1 -> Product/1  "e_Beta"
  Mux1/1 -> FIS Tree/1, Out Bus Element2/1  "FIS_In"
  Sum2/1 -> Gain4/1
  Delay/1 -> Sum2/2
  Gain/1 -> Data Type Conversion/1, Sum3/1  "Mz_yaw"
  FIS Tree/1 -> Demux/1  "FIS_Out"
  nYawRef/1 -> Sum/1
  nYaw/1 -> Sum/2
  Sum/1 -> Gain1/1  "e_Yaw"
  Data Type Conversion/1 -> Out Bus Element/1
  Data Type Conversion1/1 -> Out Bus Element1/1

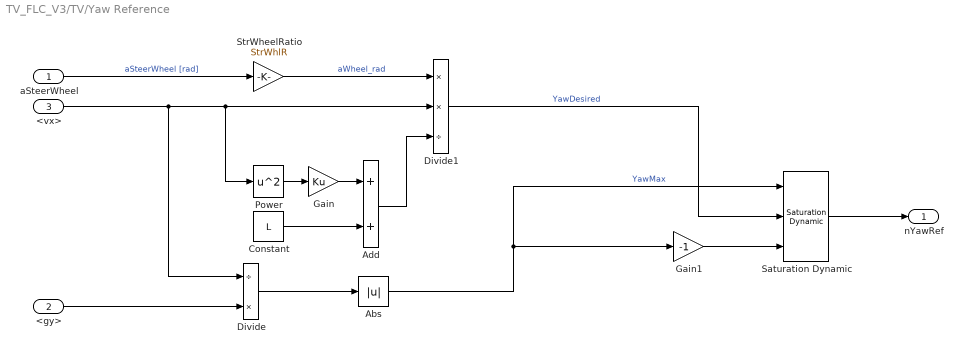
== system TV_FLC_V3/TV/Yaw Reference ==
  aSteerWheel : Inport
  <gy> : Inport  Port=2
  <vx> : Inport  Port=3
  Abs : Abs  SaturateOnIntegerOverflow=off
  Add : Sum
  Constant : Constant  Value=L  OutDataTypeStr=single
  Divide : Product  Inputs=/*
  Divide1 : Product  Inputs=**/
  Gain : Gain  Gain=Ku
  Gain1 : Gain  Gain=-1
  Power : Math  Operator=square
  Saturation Dynamic : sl_discontinuities/Saturation Dynamic  OutMin=[]  OutMax=[]  OutDataTypeStr=Inherit: Same as second input  OutDataType=fixdt(1, 16)  OutScaling=2^-10  DoSatur=off
  StrWheelRatio : Gain  Gain=StrWhlR
  nYawRef : Outport
  wires:
  Add/1 -> Divide1/3
  Constant/1 -> Add/2
  Gain/1 -> Add/1
  Power/1 -> Gain/1
  Divide1/1 -> Saturation Dynamic/2  "YawDesired"
  Gain1/1 -> Saturation Dynamic/3
  Abs/1 -> Gain1/1, Saturation Dynamic/1  "YawMax"
  Saturation Dynamic/1 -> nYawRef/1
  Divide/1 -> Abs/1
  <gy>/1 -> Divide/2
  <vx>/1 -> Divide/1, Power/1, Divide1/2
  aSteerWheel/1 -> StrWheelRatio/1  "aSteerWheel [rad]"
  StrWheelRatio/1 -> Divide1/1  "aWheel_rad"

== system TV_FLC_V3/Slip Control/Maximum Torque Allowed/Slip Correction Left ==
  kappa_rl : Inport  OutDataTypeStr=single
  Fz_rl : Inport  Port=2  OutDataTypeStr=single
  1-D Lookup Table : Lookup_n-D  NumberOfTableDimensions=1  BreakpointsForDimension1=Load_Ref  Table=Slip_Ref  ExtrapMethod=Clip  UseLastTableValue=on  InternalRulePriority=Speed  RndMeth=Simplest
  Data Type Conversion : DataTypeConversion  OutDataTypeStr=double  SaturateOnIntegerOverflow=off  RndMeth=Floor
  PID Controller : slpidlib/PID Controller  Controller=PID  Form=Parallel  TimeDomain=Discrete-time  UseExternalTs=off  SampleTime=0.003  IntegratorMethod=Forward Euler  FilterMethod=Forward Euler  ControllerParametersSource=internal  P=Slip_Ctrl_Kp  I=Slip_Ctrl_Ki  UseKiTs=off  D=Slip_Ctrl_Kd  UseExternalDerivativeSource=off  N=Slip_Ctrl_Kn  UseFilter=on  TunerSelectOption=Transfer Function Based (PID Tuner App)  InitialConditionSource=internal  InitialConditionForIntegrator=Tmax  InitialConditionForFilter=0  DifferentiatorICPrevScaledInput=Tmax  ExternalReset=none  TrackingMode=off  Kt=1  LimitOutput=on  SatLimitsSource=internal  UpperSaturationLimit=Tmax  LowerSaturationLimit=0  LinearizeAsGain=on  AntiWindupMode=clamping  Kb=1  LimitIntegrator=off  UpperIntegratorSaturationLimit=inf  LowerIntegratorSaturationLimit=-inf  POutMin=[]  POutMax=[]  IOutMin=[]  IOutMax=[]  DOutMin=[]  DOutMax=[]  NOutMin=[]  NOutMax=[]  SumOutMin=[]  SumOutMax=[]  SaturationOutMin=[]  SaturationOutMax=[]  PParamMin=[]  PParamMax=[]  IParamMin=[]  IParamMax=[]  DParamMin=[]  DParamMax=[]  NParamMin=[]  NParamMax=[]  KbParamMin=[]  KbParamMax=[]  KtParamMin=[]  KtParamMax=[]  KbOutMin=[]  KbOutMax=[]  KtOutMin=[]  KtOutMax=[]  IntegratorOutMin=[]  IntegratorOutMax=[]  FilterOutMin=[]  FilterOutMax=[]  SumI1OutMin=[]  SumI1OutMax=[]  SumI2OutMin=[]  SumI2OutMax=[]  SumI3OutMin=[]  SumI3OutMax=[]  SumI4OutMin=[]  SumI4OutMax=[]  SumDOutMin=[]  SumDOutMax=[]  DifferentiatorOutMin=[]  DifferentiatorOutMax=[]  FilterDiffOutCoefMin=[]  FilterDiffOutCoefMax=[]  ReciprocalOutMin=[]  ReciprocalOutMax=[]  SumDenOutMin=[]  SumDenOutMax=[]  SumNumOutMin=[]  SumNumOutMax=[]  DivideOutMin=[]  DivideOutMax=[]  UdiffTsProdOutMin=[]  UdiffTsProdOutMax=[]  NTsProdOutMin=[]  NTsProdOutMax=[]  UintegralTsProdOutMin=[]  UintegralTsProdOutMax=[]  UngainTsProdOutMin=[]  UngainTsProdOutMax=[]  ClampingZeroOutDataTypeStr=Inherit: Inherit via back propagation  ClampingZeroOutMin=[]  ClampingZeroOutMax=[]  FilterDenConstantOutDataTypeStr=Inherit: Inherit via back propagation  FilterDenConstantOutMin=[]  FilterDenConstantOutMax=[]  PCopyOutDataTypeStr=Inherit: Inherit via back propagation  PCopyOutMin=[]  PCopyOutMax=[]  NCopyOutDataTypeStr=Inherit: Inherit via back propagation  NCopyOutMin=[]  NCopyOutMax=[]  IntegratorContinuousStateAttributes=''  IntegratorStateMustResolveToSignalObject=off  IntegratorRTWStateStorageClass=Auto  FilterContinuousStateAttributes=''  FilterStateMustResolveToSignalObject=off  FilterRTWStateStorageClass=Auto  ParallelPVariant=InternalParameters  IdealPVariant=Disabled  IVariant=InternalParameters  DVariant=InternalParameters  IntegratorVariant=Discrete  SatVariant=Enabled  AWVariant=DiscClampingParallel  PCopyVariant=Disabled  TRVariant=Disabled  FdbkBlocksVariant=Forward  IdealPFdbkVariant=Disabled  SatFdbkVariant=Disabled  DerivativeFilterVariant=ForwardEulerFilter  NVariant=InternalParameters  NCopyVariant=Disabled  FilterICVariant=InternalICsFilter  IntegratorICVariant=InternalICs  ExternalResetVariant=Disabled  TRSumVariant=Passthrough  SumFdbkVariant=Disabled  SumVariant=Sum_PID  TsampFilterVariant=InternalTs  TsampNgainVariant=Passthrough  TsampIntegralVariant=Disabled_SignalSpec  ExternalSaturationOutDataTypeStr=Inherit: Same as second input  DerivativeSourceVariant=ErrorSignal  PreIntVariant=InternalPreInt
  Sum : Sum  Inputs=|+-
  Tmax_rl : Outport
  Out Bus Element : Outport  Port=2  PortName=Debug  Element=kappa_rl_ref
  wires:
  Data Type Conversion/1 -> Out Bus Element/1
  Fz_rl/1 -> 1-D Lookup Table/1  "Fz_rl_N"
  Sum/1 -> PID Controller/1  "e"
  1-D Lookup Table/1 -> Data Type Conversion/1, Sum/1  "kappa_ref"
  kappa_rl/1 -> Sum/2  "kappa_rl"
  PID Controller/1 -> Tmax_rl/1  "Tmax_rl_Nm"

== system TV_FLC_V3/Slip Control/Maximum Torque Allowed/Slip Correction Right ==
  Fz_rl : Inport  OutDataTypeStr=single
  kappa_rr : Inport  Port=2
  1-D Lookup Table : Lookup_n-D  NumberOfTableDimensions=1  BreakpointsForDimension1=Load_Ref  Table=Slip_Ref  ExtrapMethod=Clip  UseLastTableValue=on  InternalRulePriority=Speed  RndMeth=Simplest
  Data Type Conversion : DataTypeConversion  OutDataTypeStr=double  SaturateOnIntegerOverflow=off  RndMeth=Floor
  PID Controller : slpidlib/PID Controller  Controller=PID  Form=Parallel  TimeDomain=Discrete-time  UseExternalTs=off  SampleTime=0.003  IntegratorMethod=Forward Euler  FilterMethod=Forward Euler  ControllerParametersSource=internal  P=Slip_Ctrl_Kp  I=Slip_Ctrl_Ki  UseKiTs=off  D=Slip_Ctrl_Kd  UseExternalDerivativeSource=off  N=Slip_Ctrl_Kn  UseFilter=on  TunerSelectOption=Transfer Function Based (PID Tuner App)  InitialConditionSource=internal  InitialConditionForIntegrator=Tmax  InitialConditionForFilter=0  DifferentiatorICPrevScaledInput=Tmax  ExternalReset=none  TrackingMode=off  Kt=1  LimitOutput=on  SatLimitsSource=internal  UpperSaturationLimit=Tmax  LowerSaturationLimit=0  LinearizeAsGain=on  AntiWindupMode=clamping  Kb=1  LimitIntegrator=off  UpperIntegratorSaturationLimit=inf  LowerIntegratorSaturationLimit=-inf  POutMin=[]  POutMax=[]  IOutMin=[]  IOutMax=[]  DOutMin=[]  DOutMax=[]  NOutMin=[]  NOutMax=[]  SumOutMin=[]  SumOutMax=[]  SaturationOutMin=[]  SaturationOutMax=[]  PParamMin=[]  PParamMax=[]  IParamMin=[]  IParamMax=[]  DParamMin=[]  DParamMax=[]  NParamMin=[]  NParamMax=[]  KbParamMin=[]  KbParamMax=[]  KtParamMin=[]  KtParamMax=[]  KbOutMin=[]  KbOutMax=[]  KtOutMin=[]  KtOutMax=[]  IntegratorOutMin=[]  IntegratorOutMax=[]  FilterOutMin=[]  FilterOutMax=[]  SumI1OutMin=[]  SumI1OutMax=[]  SumI2OutMin=[]  SumI2OutMax=[]  SumI3OutMin=[]  SumI3OutMax=[]  SumI4OutMin=[]  SumI4OutMax=[]  SumDOutMin=[]  SumDOutMax=[]  DifferentiatorOutMin=[]  DifferentiatorOutMax=[]  FilterDiffOutCoefMin=[]  FilterDiffOutCoefMax=[]  ReciprocalOutMin=[]  ReciprocalOutMax=[]  SumDenOutMin=[]  SumDenOutMax=[]  SumNumOutMin=[]  SumNumOutMax=[]  DivideOutMin=[]  DivideOutMax=[]  UdiffTsProdOutMin=[]  UdiffTsProdOutMax=[]  NTsProdOutMin=[]  NTsProdOutMax=[]  UintegralTsProdOutMin=[]  UintegralTsProdOutMax=[]  UngainTsProdOutMin=[]  UngainTsProdOutMax=[]  ClampingZeroOutDataTypeStr=Inherit: Inherit via back propagation  ClampingZeroOutMin=[]  ClampingZeroOutMax=[]  FilterDenConstantOutDataTypeStr=Inherit: Inherit via back propagation  FilterDenConstantOutMin=[]  FilterDenConstantOutMax=[]  PCopyOutDataTypeStr=Inherit: Inherit via back propagation  PCopyOutMin=[]  PCopyOutMax=[]  NCopyOutDataTypeStr=Inherit: Inherit via back propagation  NCopyOutMin=[]  NCopyOutMax=[]  IntegratorContinuousStateAttributes=''  IntegratorStateMustResolveToSignalObject=off  IntegratorRTWStateStorageClass=Auto  FilterContinuousStateAttributes=''  FilterStateMustResolveToSignalObject=off  FilterRTWStateStorageClass=Auto  ParallelPVariant=InternalParameters  IdealPVariant=Disabled  IVariant=InternalParameters  DVariant=InternalParameters  IntegratorVariant=Discrete  SatVariant=Enabled  AWVariant=DiscClampingParallel  PCopyVariant=Disabled  TRVariant=Disabled  FdbkBlocksVariant=Forward  IdealPFdbkVariant=Disabled  SatFdbkVariant=Disabled  DerivativeFilterVariant=ForwardEulerFilter  NVariant=InternalParameters  NCopyVariant=Disabled  FilterICVariant=InternalICsFilter  IntegratorICVariant=InternalICs  ExternalResetVariant=Disabled  TRSumVariant=Passthrough  SumFdbkVariant=Disabled  SumVariant=Sum_PID  TsampFilterVariant=InternalTs  TsampNgainVariant=Passthrough  TsampIntegralVariant=Disabled_SignalSpec  ExternalSaturationOutDataTypeStr=Inherit: Same as second input  DerivativeSourceVariant=ErrorSignal  PreIntVariant=InternalPreInt
  Sum : Sum  Inputs=|+-
  Out Bus Element : Outport  PortName=Debug  Element=kappa_rr_ref
  Tmax_rr : Outport  Port=2
  wires:
  Data Type Conversion/1 -> Out Bus Element/1
  Fz_rl/1 -> 1-D Lookup Table/1  "Fz_rr_N"
  Sum/1 -> PID Controller/1  "e"
  kappa_rr/1 -> Sum/2  "kappa_rr"
  PID Controller/1 -> Tmax_rr/1  "Tmax_rl_Nm"
  1-D Lookup Table/1 -> Data Type Conversion/1, Sum/1  "kappa_ref"

== system TV_FLC_V3/Slip Control/Slip Calculation/Wheel Vx ==
  Vx : Inport
  nYaw : Inport  Port=2
  Add : Sum  Inputs=+-
  Add2 : Sum
  Divide : Product  Inputs=**
  Gain : Gain  Gain=1/2
  Rear Track : Constant  Value=tr  OutDataTypeStr=single
  vx_whl_rl : Outport
  vx_whl_rr : Outport  Port=2
  wires:
  Add2/1 -> vx_whl_rr/1  "vx_whl_rr"
  Add/1 -> vx_whl_rl/1  "vx_whl_rl"
  Divide/1 -> Add/2, Add2/2
  Vx/1 -> Add/1, Add2/1  "vx_m/s"
  Gain/1 -> Divide/2
  nYaw/1 -> Divide/1  "nYaw_rad/s"
  Rear Track/1 -> Gain/1  "tr_m"

== system TV_FLC_V3/TV/Yaw Moment Required/Deadband Safety ==
  e_yaw_norm : Inport
  de_yaw_norm : Inport  Port=2
  Abs de_yaw : Abs
  Abs e_yaw : Abs
  Both small : Logic  AllPortsSameDT=off  OutDataTypeStr=boolean
  Switch de_yaw : Switch  Threshold=0.5  ZeroCross=off
  Switch e_yaw : Switch  Threshold=0.5  ZeroCross=off
  Zero de_yaw : Constant  Value=0  OutDataTypeStr=single  SampleTime=0.003
  Zero e_yaw : Constant  Value=0  OutDataTypeStr=single  SampleTime=0.003
  de_yaw below deadband : simulink/Logic and Bit Operations/Compare To Constant  relop=<  const=5e-2  OutDataTypeStr=boolean  ZeroCross=off
  e_yaw below deadband : simulink/Logic and Bit Operations/Compare To Constant  relop=<  const=1e-1  OutDataTypeStr=boolean  ZeroCross=off
  e_yaw_safe : Outport
  de_yaw_safe : Outport  Port=2
  wires:
  Both small/1 -> Switch de_yaw/2, Switch e_yaw/2
  Zero e_yaw/1 -> Switch e_yaw/1
  Zero de_yaw/1 -> Switch de_yaw/1
  de_yaw below deadband/1 -> Both small/2
  e_yaw below deadband/1 -> Both small/1
  Abs e_yaw/1 -> e_yaw below deadband/1
  Switch e_yaw/1 -> e_yaw_safe/1
  Abs de_yaw/1 -> de_yaw below deadband/1
  Switch de_yaw/1 -> de_yaw_safe/1
  de_yaw_norm/1 -> Abs de_yaw/1, Switch de_yaw/3
  e_yaw_norm/1 -> Abs e_yaw/1, Switch e_yaw/3

== matlab function TV_FLC_V3/TV/Yaw Moment Required/MATLAB Function ==
  data: delta_SW input; s_turn output; delta_th parameter
function s_turn = fcn(delta_SW, delta_th)
delta_th = deg2rad(delta_th);
if delta_SW >= delta_th
    s_turn = single(+1);
elseif delta_SW <= -delta_th
    s_turn = single(-1);
elseif abs(delta_SW) < delta_th
    s_turn = single(0);
else
    s_turn = single(0);
end

end

== matlab function TV_FLC_V3/Slip Activation/MATLAB Function ==
  data: aSteerWheel input; ay input; steer_th input; nYaw input; slip_active output single; slip_active_previous input
function slip_active = fcn(aSteerWheel, ay, steer_th, nYaw,slip_active_previous)
ay_on = 0.2*9.81;
ay_off = 0.1 * 9.81;
r_on = 0.15;
r_off = 0.08;
steer_th_on = deg2rad(steer_th);
steer_th_off = deg2rad(steer_th)/2;
on_cond = abs(aSteerWheel) > steer_th_on || ...
    abs(ay)          > ay_on    || ...
    abs(nYaw)        > r_on;

off_cond = abs(aSteerWheel) < steer_th_off && ...
    abs(ay)          < ay_off    && ...
    abs(nYaw)        < r_off;

if on_cond
    slip_active = single(1);
elseif off_cond
    slip_active = single(0);
else
    slip_active = slip_active_previous;
end

end
